simulink model "boost_PID"  (R2025a)
settings: Solver=VariableStepAuto  StartTime=0.0  StopTime=10.0  RelTol=1e-3
PreLoadFcn:
  | if ~exist('Kp','var'), Kp = 0.0033193; end; if ~exist('Ki','var'), Ki = 1.41243; end; if ~exist('Kd','var'), Kd = 3.7605e-05; end; if ~exist('Nf','var'), Nf = 100; end; if ~exist('noise_sigma','var'), noise_sigma = [0 0; 1 0]; end; if ~exist('noise_Ts','var'), noise_Ts = 1e-4; end; if ~exist('noise_seed','var'), noise_seed = 23341; end
InitFcn:
  | if ~exist('Kp','var'), Kp = 0.0033193; end; if ~exist('Ki','var'), Ki = 1.41243; end; if ~exist('Kd','var'), Kd = 3.7605e-05; end; if ~exist('Nf','var'), Nf = 100; end; if ~exist('noise_sigma','var'), noise_sigma = [0 0; 1 0]; end; if ~exist('noise_Ts','var'), noise_Ts = 1e-4; end; if ~exist('noise_seed','var'), noise_seed = 23341; end
undefined symbols (not defined in the file): Kd, Ki, Kp, Nf, noise_seed, noise_Ts
libraries: spsSeriesRLCBranchLib x3, spsCurrentMeasurementLib x2, spsVoltageMeasurementLib x2, spsControlledVoltageSourceLib x1, spsDiodeLib x1, spsIGBTDiodeLib x1, spsPWMGeneratorDCDCLib x1, sps_lib x1
settings Model: Creator=Istiak  LastModifiedBy=runner

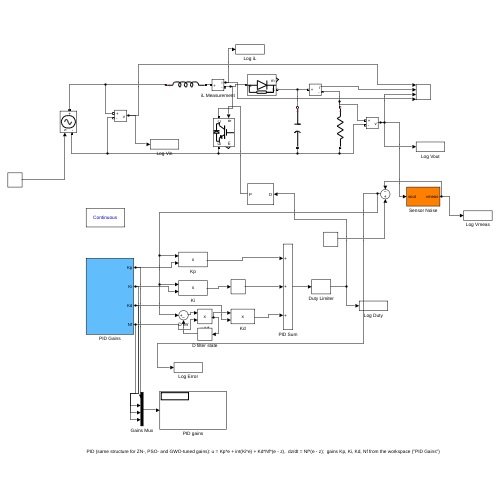
[thumbnail: Simulink's stored preview of the top-level diagram]
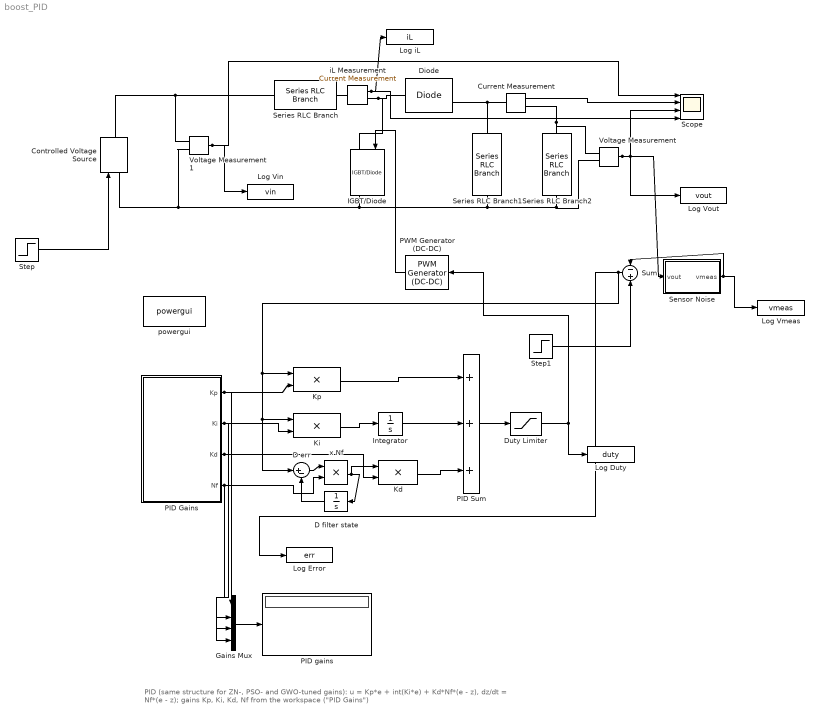
== system boost_PID ==
  note: PID (same structure for ZN-, PSO- and GWO-tuned gains): u = Kp*e + int(Ki*e) + Kd*Nf*(e - z), dz/dt = Nf*(e - z); gains Kp, Ki, Kd, Nf from the workspace ("PID Gains")
  Controlled Voltage Source : spsControlledVoltageSourceLib/Controlled Voltage Source  Initialize=on  Source_Type=AC  Amplitude=0  Phase=0  Frequency=0  Measurements=None
  Current Measurement : spsCurrentMeasurementLib/Current Measurement  PhasorSimulation=off  OutputType=Complex  PSBequivalent=0
  D err : Sum  Inputs=|+-
  D filter state : Integrator
  Diode : spsDiodeLib/Diode  Ron=0.001  Lon=0  Vf=0.8  IC=0  UseSnubber=0  Rs=500  Cs=250e-9  Measurements=on
  Duty Limiter : Saturate  UpperLimit=1  LowerLimit=0
  Gains Mux : Mux
  IGBT/Diode : spsIGBTDiodeLib/IGBT//Diode  Ron=1e-3  Rs=1e5  Cs=inf  Measurements=on
  Integrator : Integrator  LimitOutput=on  UpperSaturationLimit=1  LowerSaturationLimit=0
  Kd : Product
  Ki : Product
  Kp : Product
  Log Duty : ToWorkspace  VariableName=duty  SaveFormat=Timeseries  SampleTime=-1
  Log Error : ToWorkspace  VariableName=err  SaveFormat=Timeseries  SampleTime=-1
  Log Vin : ToWorkspace  VariableName=vin  SaveFormat=Timeseries  SampleTime=-1
  Log Vmeas : ToWorkspace  VariableName=vmeas  SaveFormat=Timeseries  SampleTime=-1
  Log Vout : ToWorkspace  VariableName=vout  SaveFormat=Timeseries  SampleTime=-1
  Log iL : ToWorkspace  VariableName=iL  SaveFormat=Timeseries  SampleTime=-1
  PID Gains : Subsystem
  PID Sum : Sum  Inputs=+++
  PID gains : Display
  PWM Generator (DC-DC) : spsPWMGeneratorDCDCLib/PWM Generator (DC-DC)  Fsw=5000  Ts=0
  Scope : Scope  NumInputPorts=4
      settings: ActiveDisplayYMinimum=11  ActiveDisplayYMaximum=21
  Sensor Noise : Subsystem
  Series RLC Branch : spsSeriesRLCBranchLib/Series RLC Branch  LConnTagsString=__new0  RConnTagsString=__new0  BranchType=L  Resistance=1  Inductance=0.0014  SetiL0=off  InitialCurrent=0  Capacitance=1e-6  Setx0=off  InitialVoltage=0  Measurements=None
  Series RLC Branch1 : spsSeriesRLCBranchLib/Series RLC Branch  LConnTagsString=__new0  RConnTagsString=__new0  BranchType=C  Resistance=1  Inductance=0.0014  SetiL0=off  InitialCurrent=0  Capacitance=0.0043  Setx0=off  InitialVoltage=0  Measurements=None
  Series RLC Branch2 : spsSeriesRLCBranchLib/Series RLC Branch  LConnTagsString=__new0  RConnTagsString=__new0  BranchType=R  Resistance=1.1520  Inductance=0.0014  SetiL0=off  InitialCurrent=0  Capacitance=0.0043  Setx0=off  InitialVoltage=0  Measurements=None
  Step : Step  Time=5  Before=12  After=20  SampleTime=0
  Step1 : Step  Before=24  After=24  SampleTime=0
  Sum : Sum  Inputs=-+
  Voltage Measurement : spsVoltageMeasurementLib/Voltage Measurement  PhasorSimulation=off  OutputType=Complex  PSBequivalent=0
  Voltage Measurement1 : spsVoltageMeasurementLib/Voltage Measurement  PhasorSimulation=off  OutputType=Complex  PSBequivalent=0
  iL Measurement : spsCurrentMeasurementLib/Current Measurement  PhasorSimulation=off  OutputType=Complex  PSBequivalent=0
  powergui : sps_lib/powergui  Priority=1  SimulationMode=Continuous  SampleTime=50e-6  frequency=60  Iterations=50  frequencyindice=0  Pbase=100e6  ErrMax=1e-4  UnitsV=kV  UnitsW=MW  buscounter=0  FunctionMessages=off  echomessages=off  EnableUseOfTLC=off  CurrentSourceSwitches=off  DisableSnubberDevices=off  DisableRonSwitches=off  DisableVfSwitches=off  DisplayEquations=off  AutomaticDiscreteSolvers=off  SolverType=Tustin/Backward Euler (TBE)  Interpol=off  ExternalGateDelay=off  methode=off  Ts=100  x0status=blocks  SPID=on  SwTol=0  HookPort=off  NonlinearTolerance=1e-4  nMaxIteration=100  ContinueOnMaxIteration=off  RestoreLinks=warning  ResistiveCurrentMeasurement=off  Frange=[0:2:500]  Ylog=off  Xlog=on  ShowGrid=off  save=off  variable=ZData  structure=0  ZoomFFT=off  StartTime=0.0  cycles=1  DisplayStyle=1  fundamental=60  FreqAxis=off  MaxFrequency=1000  frequencyindicesteady=1  RmsSteady=1  display=off
  x Nf : Product
  wires:
  Step/1 -> Controlled Voltage Source/1
  Voltage Measurement/1 -> Scope/3, Log Vout/1, Sensor Noise/1(vout)
  Step1/1 -> Sum/2
  PWM Generator (DC-DC)/1 -> IGBT/Diode/1
  Voltage Measurement1/1 -> Scope/1, Log Vin/1
  Current Measurement/1 -> Scope/2
  Sum/1 -> Ki/1, D err/1, Kp/1, Log Error/1
  Integrator/1 -> PID Sum/2
  PID Sum/1 -> Duty Limiter/1
  Duty Limiter/1 -> PWM Generator (DC-DC)/1, Log Duty/1
  Kp/1 -> PID Sum/1
  Ki/1 -> Integrator/1
  D err/1 -> x Nf/1
  x Nf/1 -> D filter state/1, Kd/1
  D filter state/1 -> D err/2
  Kd/1 -> PID Sum/3
  Gains Mux/1 -> PID gains/1
  PID Gains/1(Kp) -> Kp/2, Gains Mux/1
  PID Gains/2(Ki) -> Ki/2, Gains Mux/2
  PID Gains/3(Kd) -> Kd/2, Gains Mux/3
  PID Gains/4(Nf) -> x Nf/2, Gains Mux/4
  Sensor Noise/1(vmeas) -> Sum/1, Log Vmeas/1
  iL Measurement/1 -> Log iL/1, Scope/4
  connections:
  Series RLC Branch/LConn1 -- Voltage Measurement1/LConn1 -- Controlled Voltage Source/RConn1
  Series RLC Branch1/LConn1 -- Diode/RConn1 -- Current Measurement/LConn1
  Series RLC Branch1/RConn1 -- Voltage Measurement/LConn2 -- Series RLC Branch2/RConn1 -- Voltage Measurement1/LConn2 -- Controlled Voltage Source/LConn1 -- IGBT/Diode/RConn1
  Current Measurement/RConn1 -- Voltage Measurement/LConn1 -- Series RLC Branch2/LConn1
  Series RLC Branch/RConn1 -- iL Measurement/LConn1
  Diode/LConn1 -- iL Measurement/RConn1 -- IGBT/Diode/LConn1

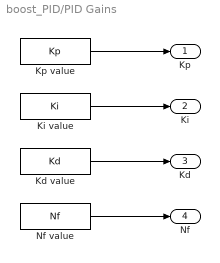
== system boost_PID/PID Gains ==
  Kd value : Constant  Value=Kd
  Ki value : Constant  Value=Ki
  Kp value : Constant  Value=Kp
  Nf value : Constant  Value=Nf
  Kp : Outport
  Ki : Outport  Port=2
  Kd : Outport  Port=3
  Nf : Outport  Port=4
  wires:
  Kp value/1 -> Kp/1
  Ki value/1 -> Ki/1
  Kd value/1 -> Kd/1
  Nf value/1 -> Nf/1

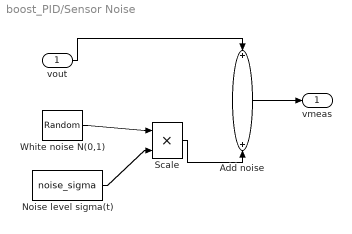
== system boost_PID/Sensor Noise ==
  vout : Inport
  Add noise : Sum
  Noise level sigma(t) : FromWorkspace  VariableName=noise_sigma  Interpolate=off  OutputAfterFinalValue=Holding final value
  Scale : Product
  White noise N(0,1) : RandomNumber  Seed=noise_seed  SampleTime=noise_Ts
  vmeas : Outport
  wires:
  White noise N(0,1)/1 -> Scale/1
  Noise level sigma(t)/1 -> Scale/2
  vout/1 -> Add noise/1
  Scale/1 -> Add noise/2
  Add noise/1 -> vmeas/1
